simulink model "afe_rst_inv_psm_distributed_control_two_delays"  (R2026a)
settings: Solver=ode1be  StopTime=simlength  FixedStep=tc  MaxStep=Tc
values from neighbouring files (symbols this model uses):
  Amplitude_U = 1.16    [grid_fault_generator.m]
  Amplitude_V = Amplitude_U    (= 1.16)    [grid_fault_generator.m]
  Amplitude_W = Amplitude_U    (= 1.16)    [grid_fault_generator.m]
  end_time_LVRT = start_time_LVRT + error_length    [grid_fault_generator.m]
  Igrid_phase_normalization_factor = 270*sqrt(2)    [grid_emulator.m]
  omega_grid_emulator_nom = w_grid    (= 314.159265359)    [grid_emulator.m]
  omega_grid_nom = w_grid    (= 314.159265359)    [grid_emulator.m]
  t_ramp = 20e-3    (= 0.02)    [grid_fault_generator.m]
  ugrid_factor = 1    [grid_emulator.m]
  V_phase_normalization_factor = Vgrid_phase_normalization_factor    [grid_emulator.m]
  Vdc_bez = 1070    [grid_emulator.m]
  Vemu_ref_norm = Vemu_ref * sqrt(2) / V_phase_normalization_factor    [grid_emulator.m]
  vn_eta_pu = 0    [grid_emulator.m]
  vn_xi_pu = 0    [grid_emulator.m]
  vp_xi_pu = 1    [grid_emulator.m]
undefined symbols (not defined in the file or in its folder): Adrso, Aresd, Bresd, CFi, CFu, Cresd, Crso, CTRPIFF_CLIP_RELEASE, dead_time_INV, emf_fb_p, emf_fb_p_ccaller_1, emf_fb_p_ccaller_2, emf_p, emf_p_ccaller_1, emf_p_ccaller_2, fPWM_INV, g0_161Hz, g0_500Hz, g1_161Hz, g1_500Hz, i_grid_neg_eta_lim, i_grid_neg_eta_red_lim, i_grid_neg_xi_lim, i_grid_neg_xi_red_lim, i_grid_pos_eta_lim, i_grid_pos_eta_red_lim, ibez, id_lim, ieta_neg_ref_lim, ieta_pos_ref_lim, iq_lim, ixi_pos_ref_lim, Jm_norm, k_frt_ref, kg, ki_afe, ki_i, ki_id, ki_iq, ki_rc_neg_grid, ki_rc_pos_grid, ki_vs, ki_w, kp_afe, kp_i, kp_id, kp_iq, kp_rc_neg_grid, kp_rc_pos_grid, kp_vs, kp_w, kw, l1, l2, Lalpha_norm, Ld_norm, Ldrso, Lq_norm, Ls_norm, luenberger_l1 ... (+30)
libraries: fl_lib x146, nesl_utility x62, simulink x8, cstblocks_lti x7, sl_discontinuities x3, single_phase_transformer_lib x3, flexshaft_lib x1, permanent_magnet_synchronous_machine x1
(part 12 of 14)

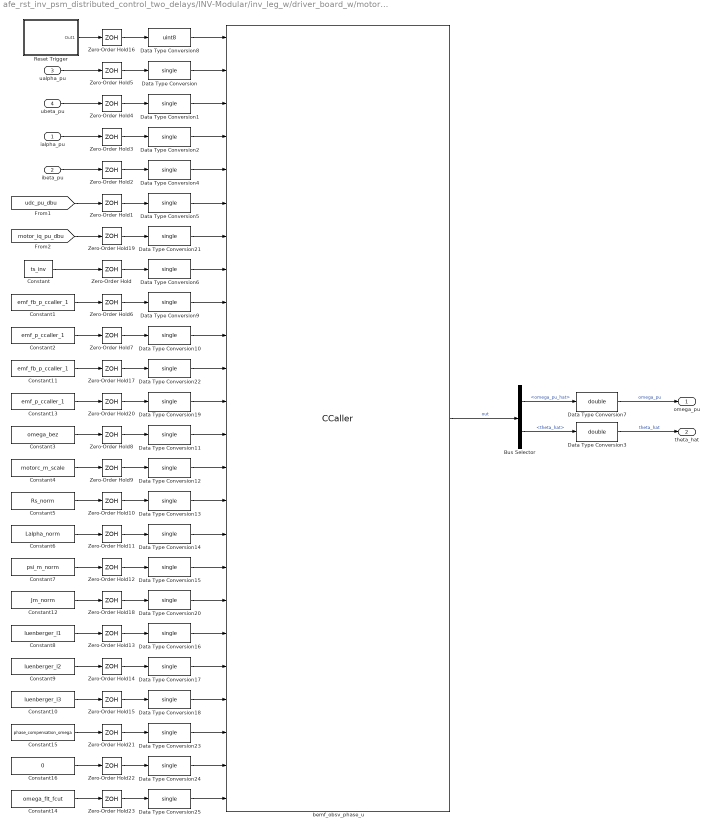
== system afe_rst_inv_psm_distributed_control_two_delays/INV-Modular/inv_leg_w/driver_board_w/motor_vector_control/bemf_observer/bemf_observer_with_load_estimator_ccaller ==
  ialpha_pu : Inport
  ibeta_pu : Inport  Port=2
  ualpha_pu : Inport  Port=3
  ubeta_pu : Inport  Port=4
  Bus Selector : BusSelector  OutputSignals=omega_pu_hat,theta_hat
  Constant : Constant  Value=ts_inv
  Constant1 : Constant  Value=emf_fb_p_ccaller_1
  Constant10 : Constant  Value=luenberger_l3
  Constant11 : Constant  Value=emf_fb_p_ccaller_1
  Constant12 : Constant  Value=Jm_norm
  Constant13 : Constant  Value=emf_p_ccaller_1
  Constant14 : Constant  Value=omega_flt_fcut
  Constant15 : Constant  Value=phase_compensation_omega
  Constant16 : Constant  Value=0
  Constant2 : Constant  Value=emf_p_ccaller_1
  Constant3 : Constant  Value=omega_bez
  Constant4 : Constant  Value=motorc_m_scale
  Constant5 : Constant  Value=Rs_norm
  Constant6 : Constant  Value=Lalpha_norm
  Constant7 : Constant  Value=psi_m_norm
  Constant8 : Constant  Value=luenberger_l1
  Constant9 : Constant  Value=luenberger_l2
  Data Type Conversion{,1..2,4..6,9..25} (23 alike) : DataTypeConversion  OutDataTypeStr=single  SaturateOnIntegerOverflow=off  RndMeth=Floor
  Data Type Conversion3 : DataTypeConversion  OutDataTypeStr=double  SaturateOnIntegerOverflow=off  RndMeth=Floor
  Data Type Conversion7 : DataTypeConversion  OutDataTypeStr=double  SaturateOnIntegerOverflow=off  RndMeth=Floor
  Data Type Conversion8 : DataTypeConversion  OutDataTypeStr=uint8  SaturateOnIntegerOverflow=off  RndMeth=Floor
  Reset Trigger : Subsystem
  Zero-Order Hold{,1..23} (24 alike) : ZeroOrderHold  SampleTime=ts_inv
  bemf_obsv_phase_u : CCaller  FunctionName=bemf_obsv_load_est_process_simulink  PortSpecificationStruct="%)30     .    (\"P   8    (     @         %    \"    !D    !     0         %  0 \"0    $    _    07)G3F%M90  4&]R=$YA;64 4V-O<&4     26YD97@     5'EP90      4VEZ90      27-';&]B86P   X    P    !@    @    $          4    (     0    ,    !         !   P!O=70 #@   #     &    \"     0         !0    @    !     P    $         $  # &]U=  .    .     8    (    !          %    \"     $    &     0         0  ...(+14838 chars)"  SampleTime=ts_inv
  omega_pu : Outport
  theta_hat : Outport  Port=2
  wires:
  Data Type Conversion5/1 -> bemf_obsv_phase_u/6
  Data Type Conversion/1 -> bemf_obsv_phase_u/2
  bemf_obsv_phase_u/1 -> Bus Selector/1  "out"
  Data Type Conversion1/1 -> bemf_obsv_phase_u/3
  Data Type Conversion4/1 -> bemf_obsv_phase_u/5
  Data Type Conversion2/1 -> bemf_obsv_phase_u/4
  Zero-Order Hold/1 -> Data Type Conversion6/1
  Zero-Order Hold5/1 -> Data Type Conversion/1
  Zero-Order Hold4/1 -> Data Type Conversion1/1
  Zero-Order Hold3/1 -> Data Type Conversion2/1
  Zero-Order Hold2/1 -> Data Type Conversion4/1
  Zero-Order Hold1/1 -> Data Type Conversion5/1
  [udc_pu_dbu] -> Zero-Order Hold1/1
  Constant/1 -> Zero-Order Hold/1
  ualpha_pu/1 -> Zero-Order Hold5/1
  ialpha_pu/1 -> Zero-Order Hold3/1
  ubeta_pu/1 -> Zero-Order Hold4/1
  ibeta_pu/1 -> Zero-Order Hold2/1
  Bus Selector/2 -> Data Type Conversion3/1  "<theta_hat>"
  Bus Selector/1 -> Data Type Conversion7/1  "<omega_pu_hat>"
  Data Type Conversion7/1 -> omega_pu/1  "omega_pu"
  Data Type Conversion3/1 -> theta_hat/1  "theta_hat"
  Reset Trigger/1(Out1) -> Zero-Order Hold16/1
  Data Type Conversion8/1 -> bemf_obsv_phase_u/1
  Constant1/1 -> Zero-Order Hold6/1
  Zero-Order Hold6/1 -> Data Type Conversion9/1
  Zero-Order Hold7/1 -> Data Type Conversion10/1
  Zero-Order Hold8/1 -> Data Type Conversion11/1
  Zero-Order Hold9/1 -> Data Type Conversion12/1
  Zero-Order Hold10/1 -> Data Type Conversion13/1
  Zero-Order Hold11/1 -> Data Type Conversion14/1
  Zero-Order Hold12/1 -> Data Type Conversion15/1
  Zero-Order Hold13/1 -> Data Type Conversion16/1
  Zero-Order Hold14/1 -> Data Type Conversion17/1
  Constant2/1 -> Zero-Order Hold7/1
  Constant3/1 -> Zero-Order Hold8/1
  Constant4/1 -> Zero-Order Hold9/1
  Constant5/1 -> Zero-Order Hold10/1
  Constant6/1 -> Zero-Order Hold11/1
  Constant7/1 -> Zero-Order Hold12/1
  Constant8/1 -> Zero-Order Hold13/1
  Constant9/1 -> Zero-Order Hold14/1
  Constant10/1 -> Zero-Order Hold15/1
  Zero-Order Hold15/1 -> Data Type Conversion18/1
  Zero-Order Hold16/1 -> Data Type Conversion8/1
  Constant12/1 -> Zero-Order Hold18/1
  Zero-Order Hold18/1 -> Data Type Conversion20/1
  Data Type Conversion6/1 -> bemf_obsv_phase_u/8
  Data Type Conversion9/1 -> bemf_obsv_phase_u/9
  Data Type Conversion10/1 -> bemf_obsv_phase_u/10
  [motor_iq_pu_dbu] -> Zero-Order Hold19/1
  Zero-Order Hold19/1 -> Data Type Conversion21/1
  Data Type Conversion21/1 -> bemf_obsv_phase_u/7
  Constant13/1 -> Zero-Order Hold20/1
  Zero-Order Hold20/1 -> Data Type Conversion19/1
  Zero-Order Hold17/1 -> Data Type Conversion22/1
  Constant11/1 -> Zero-Order Hold17/1
  Data Type Conversion22/1 -> bemf_obsv_phase_u/11
  Data Type Conversion19/1 -> bemf_obsv_phase_u/12
  Data Type Conversion11/1 -> bemf_obsv_phase_u/13
  Data Type Conversion12/1 -> bemf_obsv_phase_u/14
  Data Type Conversion13/1 -> bemf_obsv_phase_u/15
  Data Type Conversion14/1 -> bemf_obsv_phase_u/16
  Data Type Conversion15/1 -> bemf_obsv_phase_u/17
  Data Type Conversion20/1 -> bemf_obsv_phase_u/18
  Data Type Conversion16/1 -> bemf_obsv_phase_u/19
  Data Type Conversion17/1 -> bemf_obsv_phase_u/20
  Data Type Conversion18/1 -> bemf_obsv_phase_u/21
  Zero-Order Hold23/1 -> Data Type Conversion25/1
  Constant14/1 -> Zero-Order Hold23/1
  Constant16/1 -> Zero-Order Hold22/1
  Constant15/1 -> Zero-Order Hold21/1
  Zero-Order Hold22/1 -> Data Type Conversion24/1
  Zero-Order Hold21/1 -> Data Type Conversion23/1
  Data Type Conversion23/1 -> bemf_obsv_phase_u/22
  Data Type Conversion24/1 -> bemf_obsv_phase_u/23
  Data Type Conversion25/1 -> bemf_obsv_phase_u/24

== system afe_rst_inv_psm_distributed_control_two_delays/INV-Modular/inv_leg_w/driver_board_w/motor_vector_control/current_ctrl/MTPA ==
  iq : Inport
  Constant : Constant  Value=psi_m_norm
  Gain1 : Gain  Gain=1/(Lq_norm - Ld_norm)/2
  Gain2 : Gain  Gain=1/(Lq_norm - Ld_norm)/2
  Math Function1 : Math  Operator=magnitude^2  SignedPower=on
  Math Function4 : Math  Operator=magnitude^2  SignedPower=on
  Sqrt : Sqrt
  Sum : Sum  Inputs=|++
  Sum1 : Sum  Inputs=|+-
  id_ref_pu < x < 0 : Saturate  UpperLimit=0  LowerLimit=-id_lim
  Id_ref_mtpa : Outport  VectorParamsAs1DForOutWhenUnconnected=off
  wires:
  Math Function4/1 -> Sum/1
  Sum1/1 -> id_ref_pu < x < 0/1
  Constant/1 -> Gain2/1, Gain1/1
  Gain2/1 -> Sum1/1
  iq/1 -> Math Function1/1
  Sqrt/1 -> Sum1/2
  Sum/1 -> Sqrt/1
  Math Function1/1 -> Sum/2
  Gain1/1 -> Math Function4/1
  id_ref_pu < x < 0/1 -> Id_ref_mtpa/1

== system afe_rst_inv_psm_distributed_control_two_delays/INV-Modular/inv_leg_w/driver_board_w/motor_vector_control/current_ctrl/dq_pi_with_vector_antiwindup ==
  id_ref : Inport
  id : Inport  Port=2
  iq_ref : Inport  Port=3
  iq : Inport  Port=4
  dq_vector_pi : Subsystem
  dq_vector_pi_ccaller : Subsystem  Commented=on
  ctrl_d_u : Outport
  ctrl_q_u : Outport  Port=2
  wires:
  dq_vector_pi/2(ctrl_q_u) -> ctrl_q_u/1
  dq_vector_pi/1(ctrl_d_u) -> ctrl_d_u/1
  iq_ref/1 -> dq_vector_pi/4(iq_ref)  "iq_ref"
  iq/1 -> dq_vector_pi/3(iq)  "iq"
  id_ref/1 -> dq_vector_pi/2(id_ref)  "id_ref"
  id/1 -> dq_vector_pi/1(id)  "id"

== system afe_rst_inv_psm_distributed_control_two_delays/INV-Modular/inv_leg_w/driver_board_w/motor_vector_control/current_ctrl/id_ref ==
  id_mtpa : Inport
  Constant : Constant  Value=0
  Manual Switch : ManualSwitch
  id_ref : Outport
  wires:
  Constant/1 -> Manual Switch/2
  id_mtpa/1 -> Manual Switch/1
  Manual Switch/1 -> id_ref/1

== system afe_rst_inv_psm_distributed_control_two_delays/INV-Modular/inv_leg_w/modulator/sv_pwm/modulator/PWM generator ==
  m_index : Inport
  Constant : Constant  Value=dead_time*f
  Constant1 : Constant
  Data Type Conversion1 : DataTypeConversion
  Data Type Conversion2 : DataTypeConversion
  Gain : Gain  Gain=1/(pi/2)
  Gain1 : Gain  Gain=1/2
  Gain2 : Gain  Gain=vg_firing
  Gain3 : Gain  Gain=vg_firing
  Gain4 : Gain  Gain=polarity
  Gain5 : Gain  Gain=polarity
  Hit Crossing : HitCross  Commented=on  ShowOutputPort=off
  Hit Crossing1 : HitCross  Commented=on  ShowOutputPort=off
  Relational Operator1 : RelationalOperator  Operator=<=  InputSameDT=off
  Relational Operator2 : RelationalOperator  Operator=<=  InputSameDT=off
  Saturation1 : Saturate  UpperLimit=m_up  LowerLimit=m_low
  Sine Wave : Sin  Frequency=f*2*pi  Phase=-pi/2+ph  SampleTime=0
  Sum : Sum  Inputs=|++  SaturateOnIntegerOverflow=on
  Sum1 : Sum  Inputs=-+|  SaturateOnIntegerOverflow=on
  Sum2 : Sum  Inputs=|++
  Trigonometric Function1 : Trigonometry  Operator=asin
  m1 : Outport
  m2 : Outport  Port=2
  wires:
  Gain5/1 -> m2/1
  Gain4/1 -> m1/1
  Gain3/1 -> Gain5/1
  Gain2/1 -> Gain4/1
  Data Type Conversion1/1 -> Gain2/1, Hit Crossing/1
  Gain1/1 -> Relational Operator1/2, Relational Operator2/1
  Sum2/1 -> Gain1/1
  Gain/1 -> Sum2/1
  Trigonometric Function1/1 -> Gain/1
  Constant1/1 -> Sum2/2
  Sine Wave/1 -> Trigonometric Function1/1
  Sum1/1 -> Relational Operator2/2
  Sum/1 -> Relational Operator1/1
  Saturation1/1 -> Sum1/2, Sum/1
  Constant/1 -> Sum1/1, Sum/2
  Data Type Conversion2/1 -> Hit Crossing1/1, Gain3/1
  Relational Operator2/1 -> Data Type Conversion2/1
  m_index/1 -> Saturation1/1
  Relational Operator1/1 -> Data Type Conversion1/1

== system afe_rst_inv_psm_distributed_control_two_delays/AFE-Modular/afe_leg_a/driver_board_a/dq_pll/pll_stageA/sequences/alphabeta2xieta ==
  alpha : Inport
  beta : Inport  Port=2
  gamma : Inport  Port=3
  alphabeta2xieta_neg : MATLAB Function  TreatAsAtomicUnit=on  SystemSampleTime=ts_afe
  alphabeta2xieta_pos : MATLAB Function  TreatAsAtomicUnit=on  SystemSampleTime=ts_afe
  xi : Outport
  eta : Outport  Port=2
  Out3 : Outport  Port=3
  Out4 : Outport  Port=4
  wires:
  alpha/1 -> alphabeta2xieta_neg/1(alpha), alphabeta2xieta_pos/1(alpha)  "u_grid_alpha"
  beta/1 -> alphabeta2xieta_neg/2(beta), alphabeta2xieta_pos/2(beta)  "u_grid_beta"
  gamma/1 -> alphabeta2xieta_neg/3(gamma), alphabeta2xieta_pos/3(gamma)  "gamma_grid"
  alphabeta2xieta_pos/1(xi) -> xi/1  "u_grid_pos_xi"
  alphabeta2xieta_pos/2(eta) -> eta/1  "u_grid_pos_eta"
  alphabeta2xieta_neg/1(xi) -> Out3/1  "u_grid_neg_xi"
  alphabeta2xieta_neg/2(eta) -> Out4/1  "u_grid_neg_eta"

== system afe_rst_inv_psm_distributed_control_two_delays/AFE-Modular/afe_leg_a/driver_board_a/dq_pll/pll_stageA/transformation/u_500Hz_flt ==
  input : Inport
  Gain3 : Gain  Gain=g1_500Hz
  Gain6 : Gain  Gain=g0_500Hz
  Sum : Sum  Inputs=|++
  Unit Delay1 : UnitDelay  SampleTime=ts_afe
  output : Outport  VectorParamsAs1DForOutWhenUnconnected=off
  wires:
  Sum/1 -> output/1, Unit Delay1/1
  Gain3/1 -> Sum/2
  Unit Delay1/1 -> Gain3/1
  input/1 -> Gain6/1
  Gain6/1 -> Sum/1

== system afe_rst_inv_psm_distributed_control_two_delays/AFE-Modular/afe_leg_b/driver_board_b/dq_pll/pll_stageA/mormalization_and_transformation/u_500Hz_flt ==
  input : Inport
  Gain3 : Gain  Gain=g1_500Hz
  Gain6 : Gain  Gain=g0_500Hz
  Sum : Sum  Inputs=|++
  Unit Delay1 : UnitDelay  SampleTime=ts_afe
  output : Outport  VectorParamsAs1DForOutWhenUnconnected=off
  wires:
  Gain6/1 -> Sum/1
  input/1 -> Gain6/1
  Unit Delay1/1 -> Gain3/1
  Gain3/1 -> Sum/2
  Sum/1 -> Unit Delay1/1, output/1

== system afe_rst_inv_psm_distributed_control_two_delays/AFE-Modular/afe_leg_b/driver_board_b/dq_pll/pll_stageA/sequences/alphabeta2xieta ==
  alpha : Inport
  beta : Inport  Port=2
  gamma : Inport  Port=3
  alphabeta2xieta_neg : MATLAB Function  TreatAsAtomicUnit=on  SystemSampleTime=ts_afe
  alphabeta2xieta_pos : MATLAB Function  TreatAsAtomicUnit=on  SystemSampleTime=ts_afe
  xi : Outport
  eta : Outport  Port=2
  Out3 : Outport  Port=3
  Out4 : Outport  Port=4
  wires:
  alpha/1 -> alphabeta2xieta_neg/1(alpha), alphabeta2xieta_pos/1(alpha)  "u_grid_alpha"
  beta/1 -> alphabeta2xieta_neg/2(beta), alphabeta2xieta_pos/2(beta)  "u_grid_beta"
  gamma/1 -> alphabeta2xieta_neg/3(gamma), alphabeta2xieta_pos/3(gamma)  "gamma_grid"
  alphabeta2xieta_pos/1(xi) -> xi/1  "u_grid_pos_xi"
  alphabeta2xieta_pos/2(eta) -> eta/1  "u_grid_pos_eta"
  alphabeta2xieta_neg/1(xi) -> Out3/1  "u_grid_neg_xi"
  alphabeta2xieta_neg/2(eta) -> Out4/1  "u_grid_neg_eta"

== system afe_rst_inv_psm_distributed_control_two_delays/AFE-Modular/afe_leg_c/driver_board_c/dq_pll/pll_stageA/mormalization_and_transformation/u_500Hz_flt ==
  input : Inport
  Gain3 : Gain  Gain=g1_500Hz
  Gain6 : Gain  Gain=g0_500Hz
  Sum : Sum  Inputs=|++
  Unit Delay1 : UnitDelay  SampleTime=ts_afe
  output : Outport  VectorParamsAs1DForOutWhenUnconnected=off
  wires:
  Sum/1 -> output/1, Unit Delay1/1
  Gain3/1 -> Sum/2
  Unit Delay1/1 -> Gain3/1
  input/1 -> Gain6/1
  Gain6/1 -> Sum/1

== system afe_rst_inv_psm_distributed_control_two_delays/AFE-Modular/afe_leg_c/driver_board_c/dq_pll/pll_stageA/sequences/alphabeta2xieta ==
  alpha : Inport
  beta : Inport  Port=2
  gamma : Inport  Port=3
  alphabeta2xieta_neg : MATLAB Function  TreatAsAtomicUnit=on  SystemSampleTime=ts_afe
  alphabeta2xieta_pos : MATLAB Function  TreatAsAtomicUnit=on  SystemSampleTime=ts_afe
  xi : Outport
  eta : Outport  Port=2
  Out3 : Outport  Port=3
  Out4 : Outport  Port=4
  wires:
  alpha/1 -> alphabeta2xieta_neg/1(alpha), alphabeta2xieta_pos/1(alpha)  "u_grid_alpha"
  beta/1 -> alphabeta2xieta_neg/2(beta), alphabeta2xieta_pos/2(beta)  "u_grid_beta"
  gamma/1 -> alphabeta2xieta_neg/3(gamma), alphabeta2xieta_pos/3(gamma)  "gamma_grid"
  alphabeta2xieta_pos/1(xi) -> xi/1  "u_grid_pos_xi"
  alphabeta2xieta_pos/2(eta) -> eta/1  "u_grid_pos_eta"
  alphabeta2xieta_neg/1(xi) -> Out3/1  "u_grid_neg_xi"
  alphabeta2xieta_neg/2(eta) -> Out4/1  "u_grid_neg_eta"

== system afe_rst_inv_psm_distributed_control_two_delays/INV-Modular/inv_leg_u/driver_board_u/motor_vector_control/bemf_observer/bemf_observer_ccaller/Reset Trigger ==
  Step : Step  Time=0.01  InitialValue=1  FinalValue=0  SampleTime=0
  Out1 : Outport
  wires:
  Step/1 -> Out1/1  "Reset"

== system afe_rst_inv_psm_distributed_control_two_delays/INV-Modular/inv_leg_u/driver_board_u/motor_vector_control/bemf_observer/bemf_observer_simulink/double_integrator_observer ==
  theta : Inport
  Gain : Gain  Gain=kw
  Gain1 : Gain  Gain=kg
  Gain2 : Gain  Gain=omega_bez
  Gain3 : Gain  Gain=1/omega_bez
  Gain5 : Gain  Gain=ts_inv
  Sum : Sum  Inputs=-+|
  Sum1 : Sum  Inputs=|++
  Sum2 : Sum  Inputs=|++
  Sum8 : Sum  Inputs=++|
  Unit Delay1 : UnitDelay  SampleTime=ts_inv
  Unit Delay2 : UnitDelay  SampleTime=ts_inv
  bounder1 : MATLAB Function  TreatAsAtomicUnit=on  SystemSampleTime=ts_inv
  bounder2 : MATLAB Function  TreatAsAtomicUnit=on  SystemSampleTime=ts_inv
  omega_pu_hat : Outport  VectorParamsAs1DForOutWhenUnconnected=off
  theta_hat : Outport  Port=2  VectorParamsAs1DForOutWhenUnconnected=off
  tag scope: theta_hat_dbu=global
  wires:
  Unit Delay1/1 -> Sum/1, theta_hat/1, Sum2/2, [theta_hat_dbu]  "theta_hat"
  Sum/1 -> bounder1/1(u)
  Gain5/1 -> Gain2/1
  Gain3/1 -> Sum1/1
  Gain2/1 -> Sum8/1
  bounder1/1(y) -> Gain1/1, Gain/1
  bounder2/1(y) -> Unit Delay1/1
  Sum2/1 -> Sum8/2
  Unit Delay2/1 -> Gain5/1, Sum1/2, omega_pu_hat/1
  Gain/1 -> Gain3/1
  Sum1/1 -> Unit Delay2/1
  Sum8/1 -> bounder2/1(u)
  theta/1 -> Sum/2  "theta_bemf"
  Gain1/1 -> Sum2/1

== system afe_rst_inv_psm_distributed_control_two_delays/INV-Modular/inv_leg_u/driver_board_u/motor_vector_control/bemf_observer/bemf_observer_simulink/omega_hat_flt ==
  omega_hat : Inport
  Gain3 : Gain  Gain=omega_flt_g1
  Gain6 : Gain  Gain=omega_flt_g0
  Sum : Sum  Inputs=|++
  Unit Delay1 : UnitDelay  SampleTime=ts_inv
  omega_hat_flt : Outport  VectorParamsAs1DForOutWhenUnconnected=off
  wires:
  Sum/1 -> omega_hat_flt/1, Unit Delay1/1
  Gain3/1 -> Sum/2
  Unit Delay1/1 -> Gain3/1
  omega_hat/1 -> Gain6/1
  Gain6/1 -> Sum/1

== system afe_rst_inv_psm_distributed_control_two_delays/INV-Modular/inv_leg_u/driver_board_u/motor_vector_control/bemf_observer/bemf_observer_simulink/psi_alpha_hat ==
  ualpha : Inport
  ialpha : Inport  Port=2
  Gain1 : Gain  Gain=Rs_norm
  Gain2 : Gain  Gain=emf_fb_p
  Gain3 : Gain  Gain=emf_p
  Gain4 : Gain  Gain=omega_bez
  Gain5 : Gain  Gain=Ls_norm
  Gain6 : Gain  Gain=motorc_m_scale
  Gain7 : Gain  Gain=ts_inv
  Product : Product  RndMeth=Zero
  Sum : Sum  Inputs=|+-
  Sum1 : Sum  Inputs=|+-
  Sum2 : Sum  Inputs=++-  SaturateOnIntegerOverflow=on
  Sum3 : Sum  Inputs=|++
  Sum4 : Sum  Inputs=+-  SaturateOnIntegerOverflow=on
  Unit Delay1 : UnitDelay  SampleTime=ts_inv
  Unit Delay2 : UnitDelay  SampleTime=ts_inv
  psi_s_alpha_hat : Outport  VectorParamsAs1DForOutWhenUnconnected=off
  psi_r_alpha_hat : Outport  Port=2  VectorParamsAs1DForOutWhenUnconnected=off
  tag scope: psi_r_alpha_hat_dbu=global
  wires:
  Gain5/1 -> Sum4/2
  Gain6/1 -> Sum/1
  Product/1 -> Gain6/1
  Gain7/1 -> Sum3/1
  [udc_pu_dbu] -> Product/2
  Gain2/1 -> Sum2/1
  Sum1/1 -> Gain2/1
  Sum3/1 -> Unit Delay1/1  "psi_s_alpha_hat_hat"
  Unit Delay1/1 -> psi_s_alpha_hat/1, Sum4/1, Sum3/2, Gain3/1
  ualpha/1 -> Product/1
  Sum/1 -> Sum2/2
  Gain1/1 -> Sum/2
  ialpha/1 -> Gain1/1, Gain5/1
  Gain3/1 -> Sum2/3
  Sum2/1 -> Gain4/1
  Gain4/1 -> Gain7/1
  [psi_r_alpha_hat_dbu] -> Sum1/2
  [psi_r_m_alpha_dbu] -> Sum1/1
  Sum4/1 -> Unit Delay2/1
  Unit Delay2/1 -> [psi_r_alpha_hat_dbu], psi_r_alpha_hat/1

== system afe_rst_inv_psm_distributed_control_two_delays/INV-Modular/inv_leg_u/driver_board_u/motor_vector_control/bemf_observer/bemf_observer_simulink/psi_beta_hat ==
  ubeta : Inport
  ibeta : Inport  Port=2
  Gain1 : Gain  Gain=Rs_norm
  Gain2 : Gain  Gain=emf_fb_p
  Gain3 : Gain  Gain=emf_p
  Gain4 : Gain  Gain=omega_bez
  Gain5 : Gain  Gain=Ls_norm
  Gain6 : Gain  Gain=motorc_m_scale
  Gain7 : Gain  Gain=ts_inv
  Product : Product  RndMeth=Zero
  Sum : Sum  Inputs=|+-
  Sum1 : Sum  Inputs=|+-
  Sum2 : Sum  Inputs=++-  SaturateOnIntegerOverflow=on
  Sum3 : Sum  Inputs=|++
  Sum4 : Sum  Inputs=+-  SaturateOnIntegerOverflow=on
  Unit Delay1 : UnitDelay  SampleTime=ts_inv
  Unit Delay2 : UnitDelay  SampleTime=ts_inv
  psi_s_beta_hat : Outport  VectorParamsAs1DForOutWhenUnconnected=off
  psi_r_beta_hat : Outport  Port=2  VectorParamsAs1DForOutWhenUnconnected=off
  tag scope: psi_r_beta_hat_dbu=global
  wires:
  Gain5/1 -> Sum4/2
  Gain6/1 -> Sum/1
  Product/1 -> Gain6/1
  Gain7/1 -> Sum3/1
  [udc_pu_dbu] -> Product/2
  ubeta/1 -> Product/1
  Gain2/1 -> Sum2/1
  Sum3/1 -> Unit Delay1/1
  Unit Delay1/1 -> psi_s_beta_hat/1, Sum4/1, Sum3/2, Gain3/1
  [psi_r_m_beta_dbu] -> Sum1/1
  [psi_r_beta_hat_dbu] -> Sum1/2
  Sum1/1 -> Gain2/1
  Gain4/1 -> Gain7/1
  Sum2/1 -> Gain4/1
  Gain3/1 -> Sum2/3
  ibeta/1 -> Gain1/1, Gain5/1
  Gain1/1 -> Sum/2
  Sum/1 -> Sum2/2
  Sum4/1 -> Unit Delay2/1
  Unit Delay2/1 -> [psi_r_beta_hat_dbu], psi_r_beta_hat/1

== system afe_rst_inv_psm_distributed_control_two_delays/INV-Modular/inv_leg_u/driver_board_u/motor_vector_control/bemf_observer/bemf_observer_simulink/theta_bemf_hat ==
  psi_r_alpha_hat : Inport
  psi_r_beta_hat : Inport  Port=2
  omega_pu_hat : Inport  Port=3
  Sum : Sum  Inputs=|++
  Trigonometric Function : Trigonometry  Operator=atan2  OutputSignalType=real
  phase_compensation_omega : Gain  Gain=phase_compensation_omega
  theta_emf_hat : Outport  VectorParamsAs1DForOutWhenUnconnected=off
  wires:
  Sum/1 -> theta_emf_hat/1
  phase_compensation_omega/1 -> Sum/2
  omega_pu_hat/1 -> phase_compensation_omega/1
  Trigonometric Function/1 -> Sum/1
  psi_r_beta_hat/1 -> Trigonometric Function/1
  psi_r_alpha_hat/1 -> Trigonometric Function/2

== system afe_rst_inv_psm_distributed_control_two_delays/INV-Modular/inv_leg_u/driver_board_u/motor_vector_control/bemf_observer/bemf_observer_with_load_estimator_ccaller/Reset Trigger ==
  Step : Step  Time=0.01  InitialValue=1  FinalValue=0  SampleTime=0
  Out1 : Outport
  wires:
  Step/1 -> Out1/1  "Reset"

== system afe_rst_inv_psm_distributed_control_two_delays/INV-Modular/inv_leg_u/driver_board_u/motor_vector_control/current_ctrl/dq_pi_with_vector_antiwindup/dq_vector_pi ==
  id : Inport
  id_ref : Inport  Port=2
  iq : Inport  Port=3
  iq_ref : Inport  Port=4
  Sum1 : Sum  Inputs=|+-
  Sum2 : Sum  Inputs=|+-
  bounder1 : Subsystem
  bounder2 : Subsystem
  pi_d : Subsystem
  pi_q : Subsystem
  switch : Subsystem
  vector lenght : Subsystem
  ctrl_d_u : Outport
  ctrl_q_u : Outport  Port=2
  wires:
  bounder2/2(clip) -> switch/2(clip 2)
  bounder2/1(mq_sat) -> ctrl_q_u/1
  pi_q/1(Vqs_out) -> bounder2/3(mq), vector lenght/2(mq)
  vector lenght/1(m_1) -> bounder1/2(m_1), bounder2/2(m_1)
  vector lenght/2(m) -> bounder1/3(m), bounder2/1(m)
  pi_d/1(ud_out) -> vector lenght/1(md), bounder1/1(md)
  switch/1(clip) -> pi_q/2(clip), pi_d/2(clip)
  bounder1/2(clip) -> switch/1(clip 1)
  Sum2/1 -> pi_q/1(iq_tilde)
  Sum1/1 -> pi_d/1(id_tilde)
  bounder1/1(md_sat) -> ctrl_d_u/1
  id_ref/1 -> Sum1/1
  id/1 -> Sum1/2
  iq_ref/1 -> Sum2/1
  iq/1 -> Sum2/2

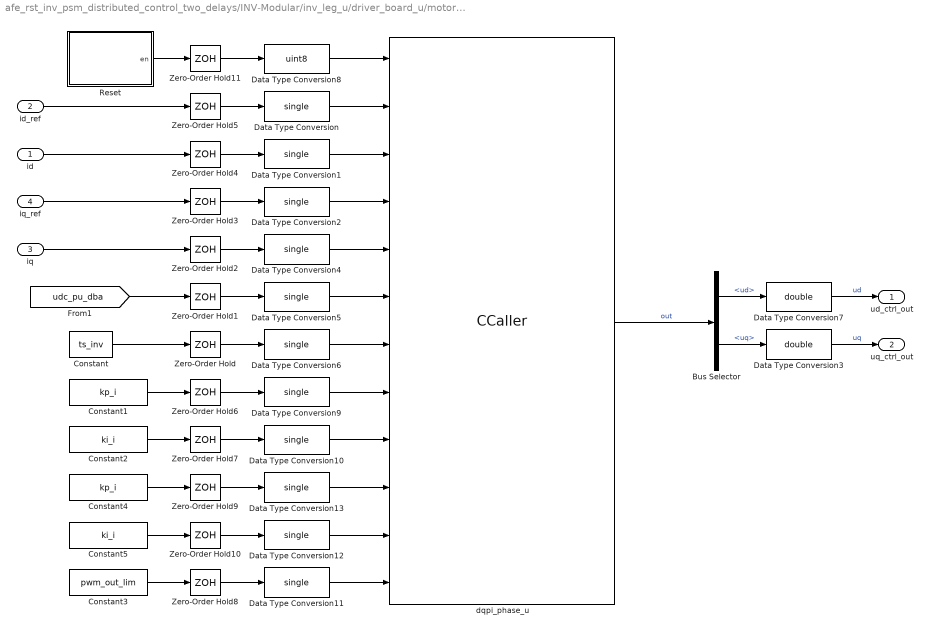
== system afe_rst_inv_psm_distributed_control_two_delays/INV-Modular/inv_leg_u/driver_board_u/motor_vector_control/current_ctrl/dq_pi_with_vector_antiwindup/dq_vector_pi_ccaller ==
  id : Inport
  id_ref : Inport  Port=2
  iq : Inport  Port=3
  iq_ref : Inport  Port=4
  Bus Selector : BusSelector  OutputSignals=ud,uq
  Constant : Constant  Value=ts_inv
  Constant1 : Constant  Value=kp_i
  Constant2 : Constant  Value=ki_i
  Constant3 : Constant  Value=pwm_out_lim
  Constant4 : Constant  Value=kp_i
  Constant5 : Constant  Value=ki_i
  Data Type Conversion{,1..2,4..6,9..13} (11 alike) : DataTypeConversion  OutDataTypeStr=single  SaturateOnIntegerOverflow=off  RndMeth=Floor
  Data Type Conversion3 : DataTypeConversion  OutDataTypeStr=double  SaturateOnIntegerOverflow=off  RndMeth=Floor
  Data Type Conversion7 : DataTypeConversion  OutDataTypeStr=double  SaturateOnIntegerOverflow=off  RndMeth=Floor
  Data Type Conversion8 : DataTypeConversion  OutDataTypeStr=uint8  SaturateOnIntegerOverflow=off  RndMeth=Floor
  Reset : Subsystem
  Zero-Order Hold{,1..11} (12 alike) : ZeroOrderHold  SampleTime=ts_inv
  dqpi_phase_u : CCaller  FunctionName=dqvector_pi_process_simulink  PortSpecificationStruct="%)30     .    ,!8   8    (     @         %    \"     T    !     0         %  0 \"0    $    _    07)G3F%M90  4&]R=$YA;64 4V-O<&4     26YD97@     5'EP90      4VEZ90      27-';&]B86P   X    P    !@    @    $          4    (     0    ,    !         !   P!O=70 #@   #     &    \"     0         !0    @    !     P    $         $  # &]U=  .    .     8    (    !          %    \"     $    &     0         0   ...(+7280 chars)"  SampleTime=ts_inv
  ud_ctrl_out : Outport
  uq_ctrl_out : Outport  Port=2
  wires:
  Data Type Conversion5/1 -> dqpi_phase_u/6
  Data Type Conversion/1 -> dqpi_phase_u/2
  dqpi_phase_u/1 -> Bus Selector/1  "out"
  Data Type Conversion1/1 -> dqpi_phase_u/3
  Data Type Conversion4/1 -> dqpi_phase_u/5
  Data Type Conversion2/1 -> dqpi_phase_u/4
  Data Type Conversion6/1 -> dqpi_phase_u/7
  Zero-Order Hold/1 -> Data Type Conversion6/1
  Zero-Order Hold5/1 -> Data Type Conversion/1
  Zero-Order Hold4/1 -> Data Type Conversion1/1
  Zero-Order Hold3/1 -> Data Type Conversion2/1
  Zero-Order Hold2/1 -> Data Type Conversion4/1
  Zero-Order Hold1/1 -> Data Type Conversion5/1
  [udc_pu_dba] -> Zero-Order Hold1/1
  Constant/1 -> Zero-Order Hold/1
  id_ref/1 -> Zero-Order Hold5/1
  iq_ref/1 -> Zero-Order Hold3/1
  id/1 -> Zero-Order Hold4/1
  iq/1 -> Zero-Order Hold2/1
  Bus Selector/2 -> Data Type Conversion3/1  "<uq>"
  Bus Selector/1 -> Data Type Conversion7/1  "<ud>"
  Data Type Conversion7/1 -> ud_ctrl_out/1  "ud"
  Data Type Conversion3/1 -> uq_ctrl_out/1  "uq"
  Reset/1(en) -> Zero-Order Hold11/1
  Data Type Conversion8/1 -> dqpi_phase_u/1
  Constant1/1 -> Zero-Order Hold6/1
  Zero-Order Hold6/1 -> Data Type Conversion9/1
  Data Type Conversion9/1 -> dqpi_phase_u/8
  Data Type Conversion10/1 -> dqpi_phase_u/9
  Zero-Order Hold7/1 -> Data Type Conversion10/1
  Zero-Order Hold8/1 -> Data Type Conversion11/1
  Constant2/1 -> Zero-Order Hold7/1
  Constant3/1 -> Zero-Order Hold8/1
  Data Type Conversion11/1 -> dqpi_phase_u/12
  Constant5/1 -> Zero-Order Hold10/1
  Zero-Order Hold10/1 -> Data Type Conversion12/1
  Zero-Order Hold9/1 -> Data Type Conversion13/1
  Constant4/1 -> Zero-Order Hold9/1
  Data Type Conversion13/1 -> dqpi_phase_u/10
  Data Type Conversion12/1 -> dqpi_phase_u/11
  Zero-Order Hold11/1 -> Data Type Conversion8/1

== system afe_rst_inv_psm_distributed_control_two_delays/INV-Modular/inv_leg_v/driver_board_v/motor_vector_control/bemf_observer/bemf_observer_ccaller/Reset Trigger ==
  Step : Step  Time=0.01  InitialValue=1  FinalValue=0  SampleTime=0
  Out1 : Outport
  wires:
  Step/1 -> Out1/1  "Reset"
